simulink model "llc_full_bridge_closed_loop"  (R2025b)
settings: Solver=ode23t  StartTime=0.0  StopTime=0.020001202000000003  MaxStep=9.9999999999999995e-08  RelTol=1.0000000000000001e-05  AbsTol=9.9999999999999995e-08
InitFcn:
  | llc_model_dir=fileparts(get_param(bdroot,'FileName'));addpath(llc_model_dir,fullfile(fileparts(llc_model_dir),'modulation'));llc_initialize_model(bdroot);
model workspace (MAT data in the model file):
  llc_control.control_period_s = 1e-05
  llc_control.voltage_filter_time_constant_s = 5e-05
  llc_control.reference_ramp_time_s = 0.001
  llc_control.reference_voltage_v = 48
  llc_control.initial_frequency_hz = 180000
  llc_control.bias_frequency_hz = 110000
  llc_control.frequency_slew_rate_hz_per_s = 100000000
  llc_control.proportional_gain_hz_per_v = 1000
  llc_control.integral_gain_hz_per_v_s = 5000000
  llc_control.deadtime_s = 2e-07
  llc_control.minimum_pulse_s = 5e-07
  llc_events.gate_times_s = [0 2e-07 2.5e-06 2.7e-06 5e-06 5.2e-06 7.5e-06 7.7e-06 1e-05 1.02e-05 1.25e-05 1.27e-05 ... (8813 elements, 8813x1)]
  llc_events.gate_values = [0 1 0 0 0 1 0 0 0 1 0 0 ... (35248 elements, 8812x4)]
  llc_events.cycle_times_s = [0 5e-06 1e-05 1.5e-05 2e-05 2.5e-05 3e-05 3.5e-05 4e-05 4.5e-05 5e-05 5.5e-05 ... (2203 elements, 2203x1)]
  llc_events.requested_frequency_hz = [200000 200000 200000 200000 200000 200000 200000 200000 200000 200000 200000 200000 ... (2203 elements, 2203x1)]
  llc_events.actual_frequency_hz = [200000 200000 200000 200000 200000 200000 200000 200000 200000 200000 200000 200000 ... (2203 elements, 2203x1)]
  llc_events.stop_time_s = 0.020001202
  llc_events.actual_step_time_s = 0.015001702
  llc_events.gate_source = timeseries
  llc_events.gate_source.Name = 'unnamed'
  llc_events.gate_source.DataInfo = tsdata.datametadata
  llc_events.gate_source.DataInfo.Interpolation = tsdata.interpolation
  llc_events.gate_source.DataInfo.Interpolation.Fhandle : function handle (value not decoded)
  llc_events.gate_source.DataInfo.Interpolation.Name = 'zoh'
  llc_events.gate_source.TimeInfo = tsdata.timemetadata
  llc_events.gate_source.TimeInfo.Length = 8813
  llc_events.gate_source.TimeInfo.DuplicateTimes = 0
  llc_events.gate_source.TimeInfo.Time_ = [0 2e-07 2.5e-06 2.7e-06 5e-06 5.2e-06 7.5e-06 7.7e-06 1e-05 1.02e-05 1.25e-05 1.27e-05 ... (8813 elements, 8813x1)]
  llc_events.gate_source.TimeInfo.Initialized = 1
  llc_events.gate_source.QualityInfo = tsdata.qualmetadata
  llc_events.gate_source.Data_ = [0 1 0 0 0 1 0 0 0 1 0 0 ... (35252 elements, 8813x4)]
  llc_excitation.start_time_s = 0
  llc_excitation.envelope_rise_time_s = 0
  llc_excitation.vin.center_value = 400
  llc_excitation.vin.amplitude = 0
  llc_excitation.vin.frequency_hz = 0
  llc_excitation.vin.phase_rad = 0
  llc_excitation.reference.center_value = 48
  llc_excitation.reference.amplitude = 0
  llc_excitation.reference.frequency_hz = 0
  llc_excitation.reference.phase_rad = 0
  llc_gate_source = timeseries
  llc_gate_source.Name = 'unnamed'
  llc_gate_source.DataInfo = tsdata.datametadata
  llc_gate_source.DataInfo.Interpolation = tsdata.interpolation
  llc_gate_source.DataInfo.Interpolation.Fhandle : function handle (value not decoded)
  llc_gate_source.DataInfo.Interpolation.Name = 'zoh'
  llc_gate_source.TimeInfo = tsdata.timemetadata
  llc_gate_source.TimeInfo.Length = 8813
  llc_gate_source.TimeInfo.DuplicateTimes = 0
  llc_gate_source.TimeInfo.Time_ = [0 2e-07 2.5e-06 2.7e-06 5e-06 5.2e-06 7.5e-06 7.7e-06 1e-05 1.02e-05 1.25e-05 1.27e-05 ... (8813 elements, 8813x1)]
  llc_gate_source.TimeInfo.Initialized = 1
  llc_gate_source.QualityInfo = tsdata.qualmetadata
  llc_gate_source.Data_ = [0 1 0 0 0 1 0 0 0 1 0 0 ... (35252 elements, 8813x4)]
  llc_p.design_id = 'llc-400v-48v-1kw-candidate-01'
  llc_p.status = 'candidate_not_hardware_validated'
  llc_p.parameter_basis = 'Analytical FHA sizing and explicit simulation assumptions; not measured device data'
  llc_p.vin_v = 400
  llc_p.vin_range_v = [360; 440]
  llc_p.output_target_v = 48
  llc_p.power_target_w = 1000
  llc_p.load_ohm = 2.304
  llc_p.turns_ratio_np_ns = 8
  llc_p.resonant_inductance_h = 7.6e-05
  llc_p.resonant_capacitance_f = 3.3e-08
  llc_p.magnetizing_inductance_h = 0.00038
  llc_p.output_capacitance_f = 0.001
  llc_p.resonant_winding_resistance_ohm = 0.1
  llc_p.magnetizing_series_resistance_ohm = 0.1
  llc_p.switch_on_resistance_ohm = 0.08
  llc_p.switch_off_conductance_s = 1e-08
  llc_p.body_diode_forward_v = 0.8
  llc_p.body_diode_on_resistance_ohm = 0.02
  llc_p.rectifier_forward_v = 0.6
  llc_p.rectifier_on_resistance_ohm = 0.005
  llc_p.diode_off_conductance_s = 1e-08
  llc_p.deadtime_s = 2e-07
  llc_p.minimum_pulse_s = 5e-07
  llc_p.time_tick_s = 1e-09
  llc_p.frequency_range_hz = [70000; 220000]
  llc_p.startup_frequency_hz = 200000
  llc_p.nominal_frequency_hz = 102000
  llc_p.step_frequency_hz = 110000
  llc_p.startup_hold_s = 0.0005
  llc_p.startup_ramp_end_s = 0.002
  llc_p.frequency_step_request_s = 0.015
  llc_p.stop_request_s = 0.02
  llc_p.max_step_s = 1e-07
  llc_p.relative_tolerance = 1e-05
  llc_p.absolute_tolerance = 1e-07
  llc_p.state_names = {'i_Lr'; 'v_Cr'; 'i_Lm'; 'v_o'}
  llc_p.state_units = {'A'; 'V'; 'A'; 'V'}
  llc_p.gate_names = {'Q1_A_high'; 'Q2_A_low'; 'Q3_B_high'; 'Q4_B_low'}
  llc_p.resonant_frequency_hz = 100497.756231
  llc_p.config_file = '\\wsl.localhost\ubuntu-22.04\home\antep\projects\LLC_Neural_ODE\configs\llc_candidate.json'
  llc_refinement = 1
libraries: fl_lib x25, nesl_utility x10
settings Model: Creator=antep  LastModifiedBy=antep

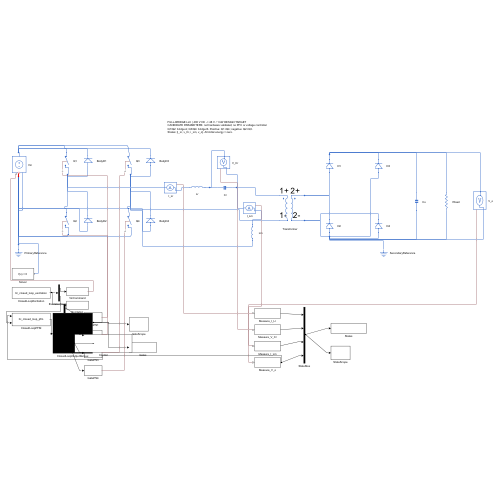
[thumbnail: Simulink's stored preview of the top-level diagram]
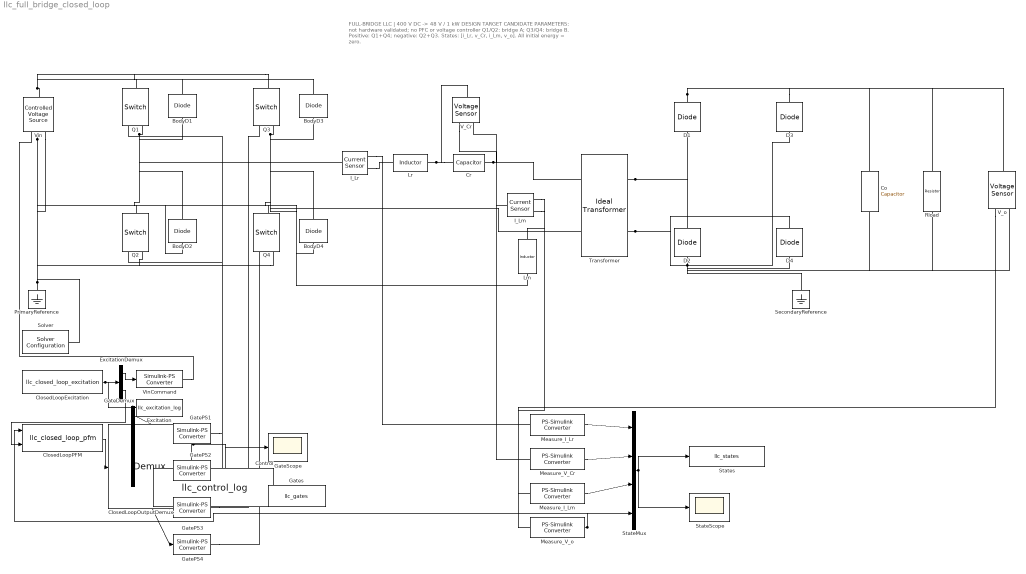
== system llc_full_bridge_closed_loop ==
  note: FULL-BRIDGE LLC | 400 V DC -> 48 V / 1 kW DESIGN TARGET
      | CANDIDATE PARAMETERS: not hardware validated; no PFC or voltage controller
      | Q1/Q2: bridge A; Q3/Q4: bridge B. Positive: Q1+Q4; negative: Q2+Q3.
      | States: [i_Lr, v_Cr, i_Lm, v_o]. All initial energy = zero.
  BodyD{1..4} (4 alike) : fl_lib/Electrical/Electrical Elements/Diode  Vf=llc_p.body_diode_forward_v V  Ron=llc_p.body_diode_on_resistance_ohm Ohm  Goff=llc_p.diode_off_conductance_s 1/Ohm  i_specify=off  i_priority=None  i=0 A  i_nominal_specify=off  i_nominal_value=1  i_nominal_unit=A  v_specify=off  v_priority=None  v=0 V  v_nominal_specify=off  v_nominal_value=1  v_nominal_unit=V
  ClosedLoopExcitation : M-S-Function  FunctionName=llc_closed_loop_excitation  Parameters=llc_excitation
  ClosedLoopOutputDemux : Demux  Outputs=[4 5]
  ClosedLoopPFM : M-S-Function  FunctionName=llc_closed_loop_pfm  Parameters=llc_control
  Co : fl_lib/Electrical/Electrical Elements/Capacitor  c=llc_p.output_capacitance_f F  r=0 Ohm  g=0 1/Ohm  i_specify=off  i_priority=None  i=0 A  i_nominal_specify=off  i_nominal_value=1  i_nominal_unit=A  v_specify=off  v_priority=None  v=0 V  v_nominal_specify=off  v_nominal_value=1  v_nominal_unit=V  vc_specify=on  vc_priority=High  vc=0 V  vc_nominal_specify=off  vc_nominal_value=1  vc_nominal_unit=V
  Control : ToWorkspace  VariableName=llc_control_log  SaveFormat=Timeseries  SampleTime=-1
  Cr : fl_lib/Electrical/Electrical Elements/Capacitor  c=llc_p.resonant_capacitance_f F  r=0 Ohm  g=0 1/Ohm  i_specify=off  i_priority=None  i=0 A  i_nominal_specify=off  i_nominal_value=1  i_nominal_unit=A  v_specify=off  v_priority=None  v=0 V  v_nominal_specify=off  v_nominal_value=1  v_nominal_unit=V  vc_specify=on  vc_priority=High  vc=0 V  vc_nominal_specify=off  vc_nominal_value=1  vc_nominal_unit=V
  D{1..4} (4 alike) : fl_lib/Electrical/Electrical Elements/Diode  Vf=llc_p.rectifier_forward_v V  Ron=llc_p.rectifier_on_resistance_ohm Ohm  Goff=llc_p.diode_off_conductance_s 1/Ohm  i_specify=off  i_priority=None  i=0 A  i_nominal_specify=off  i_nominal_value=1  i_nominal_unit=A  v_specify=off  v_priority=None  v=0 V  v_nominal_specify=off  v_nominal_value=1  v_nominal_unit=V
  Excitation : ToWorkspace  VariableName=llc_excitation_log  SaveFormat=Timeseries  SampleTime=-1
  ExcitationDemux : Demux  Outputs=2
  GateDemux : Demux
  GatePS{1..4} (4 alike) : nesl_utility/Simulink-PS Converter  PhysicalDomain=network_engine_domain  SubClassName=ps_input  LeftPortType=input  RightPortType=output  PseudoPeriodic=off  Frequencies=[]  NoiseDistribution=none  NoiseParameters=[]  Unit=1  AffineConversion=off  FilteringAndDerivatives=provide  SimscapeFilterOrder=1  InputFilterTimeConstant=0.001  UdotUserProvided=0
  GateScope : Scope
  Gates : ToWorkspace  VariableName=llc_gates  SaveFormat=Timeseries  SampleTime=-1
  I_Lm : fl_lib/Electrical/Electrical Sensors/Current Sensor
  I_Lr : fl_lib/Electrical/Electrical Sensors/Current Sensor
  Lm : fl_lib/Electrical/Electrical Elements/Inductor  l=llc_p.magnetizing_inductance_h H  r=llc_p.magnetizing_series_resistance_ohm Ohm  g=0 1/Ohm  i_specify=off  i_priority=None  i=0 A  i_nominal_specify=off  i_nominal_value=1  i_nominal_unit=A  v_specify=off  v_priority=None  v=0 V  v_nominal_specify=off  v_nominal_value=1  v_nominal_unit=V  i_L_specify=on  i_L_priority=High  i_L=0 A  i_L_nominal_specify=off  i_L_nominal_value=1  i_L_nominal_unit=A
  Lr : fl_lib/Electrical/Electrical Elements/Inductor  l=llc_p.resonant_inductance_h H  r=llc_p.resonant_winding_resistance_ohm Ohm  g=0 1/Ohm  i_specify=off  i_priority=None  i=0 A  i_nominal_specify=off  i_nominal_value=1  i_nominal_unit=A  v_specify=off  v_priority=None  v=0 V  v_nominal_specify=off  v_nominal_value=1  v_nominal_unit=V  i_L_specify=on  i_L_priority=High  i_L=0 A  i_L_nominal_specify=off  i_L_nominal_value=1  i_L_nominal_unit=A
  Measure_I_Lm : nesl_utility/PS-Simulink Converter  PhysicalDomain=network_engine_domain  SubClassName=ps_output  LeftPortType=input  RightPortType=output  PseudoPeriodic=off  Frequencies=[]  VectorFormat=inherit  Unit=A  AffineConversion=off
  Measure_I_Lr : nesl_utility/PS-Simulink Converter  PhysicalDomain=network_engine_domain  SubClassName=ps_output  LeftPortType=input  RightPortType=output  PseudoPeriodic=off  Frequencies=[]  VectorFormat=inherit  Unit=A  AffineConversion=off
  Measure_V_Cr : nesl_utility/PS-Simulink Converter  PhysicalDomain=network_engine_domain  SubClassName=ps_output  LeftPortType=input  RightPortType=output  PseudoPeriodic=off  Frequencies=[]  VectorFormat=inherit  Unit=V  AffineConversion=off
  Measure_V_o : nesl_utility/PS-Simulink Converter  PhysicalDomain=network_engine_domain  SubClassName=ps_output  LeftPortType=input  RightPortType=output  PseudoPeriodic=off  Frequencies=[]  VectorFormat=inherit  Unit=V  AffineConversion=off
  PrimaryReference : fl_lib/Electrical/Electrical Elements/Electrical Reference
  Q{1..4} (4 alike) : fl_lib/Electrical/Electrical Elements/Switch  R_closed=llc_p.switch_on_resistance_ohm Ohm  G_open=llc_p.switch_off_conductance_s 1/Ohm  Threshold=0.5  i_specify=off  i_priority=None  i=0 A  i_nominal_specify=off  i_nominal_value=1  i_nominal_unit=A  v_specify=off  v_priority=None  v=0 V  v_nominal_specify=off  v_nominal_value=1  v_nominal_unit=V
  Rload : fl_lib/Electrical/Electrical Elements/Resistor  R=llc_p.load_ohm Ohm  i_specify=off  i_priority=None  i=0 A  i_nominal_specify=off  i_nominal_value=1  i_nominal_unit=A  v_specify=off  v_priority=None  v=0 V  v_nominal_specify=off  v_nominal_value=1  v_nominal_unit=V
  SecondaryReference : fl_lib/Electrical/Electrical Elements/Electrical Reference
  Solver : nesl_utility/Solver Configuration  PhysicalDomain=network_engine_domain  SubClassName=solver  LeftPortType=input  RightPortType=generic  Tones=[]  Harmonics=[]  SimulateNoise=off  Profile=off  UseLocalSampling=off  EnableSwitchedLinearOptims=on  FrequencyDomain=off  UseCCode=off  RelTol=0.001  AbsTol=0.001  MinStep=1e-09  ToWorkspace=off  RevertToSquareIcSolve=off  NumHomotopyIterations=100  PhasorMode=off  PhasorModeNumHarmonics=1  ConsistencySolver=NEWTON_XTOL_AFTER_FTOL  IndexReductionMethod=DerivativeReplacement  DoDC=off  ResidualTolerance=1e-09  ConsistencyTolSource=GLOBAL  ConsistencyAbsTol=0.001  ConsistencyRelTol=0.001  ConsistencyTolFactor=0.001  UseLocalSolver=off  LocalSolverChoice=NE_BACKWARD_EULER_ADVANCER  ResolveIndetEquations=on  FunctionEvalNumThread=1  LocalSolverSampleTime=0.001  DoFixedCost=off  MaxNonlinIter=3  MaxModeIter=2  ComputeImpulses=off  ImpulseIterations=2  LinearAlgebra=auto  LinearAlgebraNumThread=0  EquationFormulation=NE_TIME_EF  DelaysMemoryBudget=1024  AutomaticFiltering=on  FilteringTimeConstant=0.001  PartitionStorageMethod=AS_NEEDED  PartitionMemoryBudget=1024  PartitionMethod=ROBUST  MultibodyUseLocalSolver=off  MultibodyLocalSolverChoice=ODE1  MultibodyLocalSolverSampleTime=0.001
  StateMux : Mux
  StateScope : Scope
  States : ToWorkspace  VariableName=llc_states  SaveFormat=Timeseries  SampleTime=-1
  Transformer : fl_lib/Electrical/Electrical Elements/Ideal Transformer  n=llc_p.turns_ratio_np_ns  i1_specify=off  i1_priority=None  i1=0 A  i1_nominal_specify=off  i1_nominal_value=1  i1_nominal_unit=A  v1_specify=off  v1_priority=None  v1=0 V  v1_nominal_specify=off  v1_nominal_value=1  v1_nominal_unit=V  i2_specify=off  i2_priority=None  i2=0 A  i2_nominal_specify=off  i2_nominal_value=1  i2_nominal_unit=A  v2_specify=off  v2_priority=None  v2=0 V  v2_nominal_specify=off  v2_nominal_value=1  v2_nominal_unit=V
  V_Cr : fl_lib/Electrical/Electrical Sensors/Voltage Sensor
  V_o : fl_lib/Electrical/Electrical Sensors/Voltage Sensor
  Vin : fl_lib/Electrical/Electrical Sources/Controlled Voltage Source
  VinCommand : nesl_utility/Simulink-PS Converter  PhysicalDomain=network_engine_domain  SubClassName=ps_input  LeftPortType=input  RightPortType=output  PseudoPeriodic=off  Frequencies=[]  NoiseDistribution=none  NoiseParameters=[]  Unit=V  AffineConversion=off  FilteringAndDerivatives=zero  SimscapeFilterOrder=1  InputFilterTimeConstant=0.001  UdotUserProvided=0
  wires:
  GateDemux/1 -> GatePS1/1
  GateDemux/2 -> GatePS2/1
  GateDemux/3 -> GatePS3/1
  GateDemux/4 -> GatePS4/1
  Measure_I_Lr/1 -> StateMux/1
  Measure_V_Cr/1 -> StateMux/2
  Measure_I_Lm/1 -> StateMux/3
  Measure_V_o/1 -> StateMux/4, ClosedLoopPFM/1
  StateMux/1 -> States/1, StateScope/1
  ClosedLoopExcitation/1 -> ExcitationDemux/1, Excitation/1
  ExcitationDemux/2 -> ClosedLoopPFM/2
  ExcitationDemux/1 -> VinCommand/1
  ClosedLoopPFM/1 -> ClosedLoopOutputDemux/1
  ClosedLoopOutputDemux/1 -> GateDemux/1, Gates/1, GateScope/1
  ClosedLoopOutputDemux/2 -> Control/1
  connections:
  Q1/LConn1 -- Vin/LConn1 -- Q3/LConn1 -- BodyD1/RConn1 -- BodyD3/RConn1
  Q2/RConn2 -- Q4/RConn2 -- BodyD2/LConn1 -- BodyD4/LConn1 -- Solver/RConn1 -- PrimaryReference/LConn1 -- Vin/RConn2
  Q2/LConn1 -- Q1/RConn2 -- BodyD1/LConn1 -- BodyD2/RConn1 -- I_Lr/LConn1
  Q4/LConn1 -- Q3/RConn2 -- BodyD3/LConn1 -- BodyD4/RConn1 -- Lm/RConn1 -- Transformer/LConn2
  I_Lr/RConn2 -- Lr/LConn1
  Cr/LConn1 -- Lr/RConn1 -- V_Cr/LConn1
  V_Cr/RConn2 -- Cr/RConn1 -- I_Lm/LConn1 -- Transformer/LConn1
  I_Lm/RConn2 -- Lm/LConn1
  D1/LConn1 -- Transformer/RConn1 -- D2/RConn1
  D3/LConn1 -- Transformer/RConn2 -- D4/RConn1
  D3/RConn1 -- D1/RConn1 -- Co/LConn1 -- Rload/LConn1 -- V_o/LConn1
  D4/LConn1 -- D2/LConn1 -- Co/RConn1 -- Rload/RConn1 -- V_o/RConn2 -- SecondaryReference/LConn1
  GatePS1/RConn1 -- Q1/RConn1
  GatePS2/RConn1 -- Q2/RConn1
  GatePS3/RConn1 -- Q3/RConn1
  GatePS4/RConn1 -- Q4/RConn1
  I_Lr/RConn1 -- Measure_I_Lr/LConn1
  V_Cr/RConn1 -- Measure_V_Cr/LConn1
  I_Lm/RConn1 -- Measure_I_Lm/LConn1
  V_o/RConn1 -- Measure_V_o/LConn1
  VinCommand/RConn1 -- Vin/RConn1
